simulink model "adrc_pid"  (R2025b)
settings: Solver=VariableStepAuto  StartTime=0.0  StopTime=50  RelTol=1e-3
values from neighbouring files (symbols this model uses):
  Alloc = [ kf,     kf,     kf,     kf ... (first row only)    [quad_params.m]
  Area = 2*L*Width    (= 0.072)    [quad_params.m]
  g = 9.81    [quad_params.m]
  h = [0 ... (first row only)    [Madgwick.m]    (also in quad_params.m = 0.2; umich_learning.m = x(:,1))
  h0 = Ts    (= 0.001)    [quad_params.m]
  inertia_mx = [Ixx; Iyy; Izz;]    [quad_params.m]
  init_h = 0.03    [quad_params.m]
  K_alloc = Alloc \ diag([W, 1, 1, 1])    [quad_params.m]
  max_rad_s_2 = max_rad_s ^ 2    (= 4279618.17072)    [quad_params.m]
  r0_position = 1    [quad_params.m]
  rho_air = 1.225    [quad_params.m]
  rho_water = 1000    [quad_params.m]
  Trot = 0.01    [quad_params.m]
  Ts = 0.001    [get_noise.m]    (also in quad_params.m; test.m = 0.002)
  W = 0.7 + 4*m_prop    (= 0.74)    [quad_params.m]
undefined symbols (not defined in the file or in its folder): adrcD
libraries: simulink x8
settings Model: Creator=David  LastModifiedBy=David

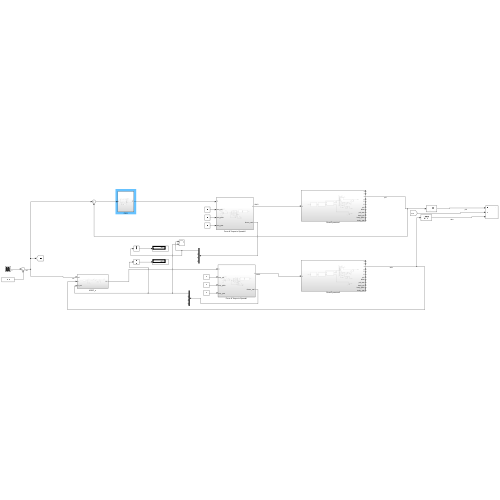
[thumbnail: Simulink's stored preview of the top-level diagram]
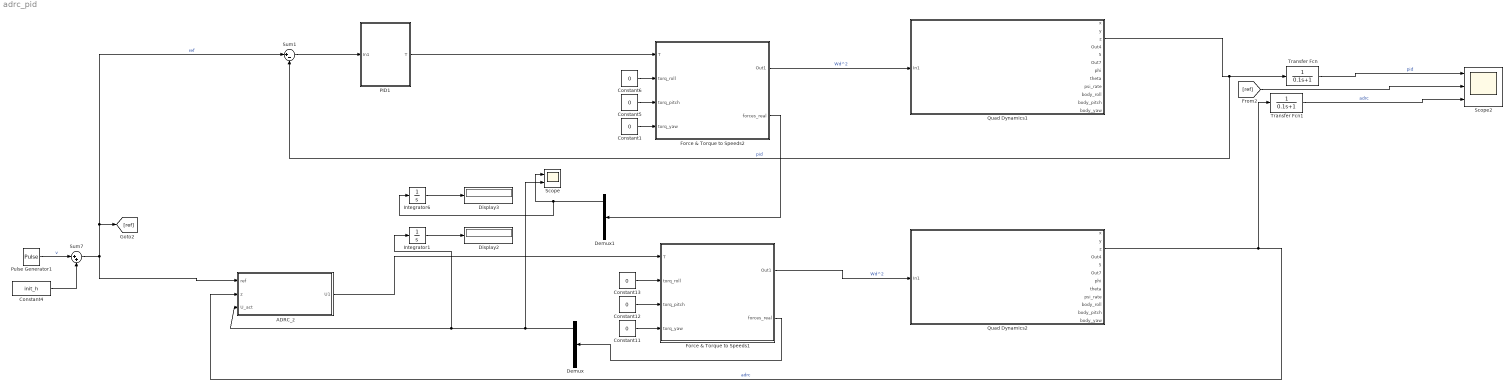
== system adrc_pid ==
  ADRC_z : Subsystem
  Constant{1,5..6,11..13} (6 alike) : Constant  Value=0
  Constant4 : Constant  Value=init_h
  Demux : Demux
  Demux1 : Demux
  Display2 : Display
  Display3 : Display
  Force & Torque to Speeds1 : Subsystem
  Force & Torque to Speeds2 : Subsystem
  Integrator1 : Integrator
  Integrator6 : Integrator
  PID1 : Subsystem
  Pulse Generator1 : DiscretePulseGenerator  PulseType=Time based  Period=30  PulseWidth=50  PhaseDelay=2
  Quad Dynamics1 : Subsystem
  Quad Dynamics2 : Subsystem
  Scope : Scope  NumInputPorts=2
      settings: ActiveDisplayYMinimum=-3.3627043852616136  ActiveDisplayYMaximum=30.264339467354532
  Scope2 : Scope  NumInputPorts=3
      settings: ActiveDisplayYMinimum=-0.12874999999999998  ActiveDisplayYMaximum=1.15875  DataLoggingVariableName=ScopeData2
  Sum1 : Sum  Inputs=|+-
  Sum7 : Sum  Inputs=|++
  Transfer Fcn : TransferFcn  Denominator=[0.1 1]
  Transfer Fcn1 : TransferFcn  Denominator=[0.1 1]
  wires:
  Integrator6/1 -> Display3/1
  Integrator1/1 -> Display2/1
  Pulse Generator1/1 -> Sum7/1  "v"
  ADRC_z/1(U1) -> Force & Torque to Speeds1/1(T)
  Constant4/1 -> Sum7/2
  Sum7/1 -> ADRC_z/1(ref), [ref], Sum1/1  "ref"
  Sum1/1 -> PID1/1(In1)
  PID1/1(T) -> Force & Torque to Speeds2/1(T)
  Constant11/1 -> Force & Torque to Speeds1/4(torq_yaw)
  Constant12/1 -> Force & Torque to Speeds1/3(torq_pitch)
  Constant13/1 -> Force & Torque to Speeds1/2(torq_roll)
  Quad Dynamics2/3(z) -> ADRC_z/2(z), Transfer Fcn1/1  "adrc"
  Constant1/1 -> Force & Torque to Speeds2/4(torq_yaw)
  Constant5/1 -> Force & Torque to Speeds2/3(torq_pitch)
  Constant6/1 -> Force & Torque to Speeds2/2(torq_roll)
  [ref] -> Scope2/2
  Force & Torque to Speeds2/1(Out1) -> Quad Dynamics1/1(In1)  "Wd^2"
  Force & Torque to Speeds1/1(Out1) -> Quad Dynamics2/1(In1)  "Wd^2"
  Force & Torque to Speeds1/2(forces_real) -> Demux/1
  Demux/1 -> Scope/2, Integrator1/1, ADRC_z/3(U_act)
  Quad Dynamics1/3(z) -> Sum1/2, Transfer Fcn/1  "pid"
  Transfer Fcn/1 -> Scope2/1  "pid"
  Transfer Fcn1/1 -> Scope2/3  "adrc"
  Force & Torque to Speeds2/2(forces_real) -> Demux1/1
  Demux1/1 -> Integrator6/1, Scope/1

== system adrc_pid/ADRC_z ==
  ref : Inport
  z : Inport  Port=2
  U_act : Inport  Port=3
  Constant : Constant  Value=adrcD.z.b0
  Constant1 : Constant  Commented=on  Value=g
  Divide : Product  Inputs=*/
  Gain : Gain  Gain=adrcD.z.k1
  Gain1 : Gain  Gain=1/W
  Gain2 : Gain  Gain=adrcD.z.k2
  Scope : Scope
      settings: ActiveDisplayYMinimum=-1  ActiveDisplayYMaximum=1  DataLoggingVariableName=ScopeData24
  Scope1 : Scope
      settings: ActiveDisplayYMinimum=-1  ActiveDisplayYMaximum=1  DataLoggingVariableName=ScopeData7
  Scope3 : Scope
      settings: ActiveDisplayYMinimum=-1  ActiveDisplayYMaximum=1  DataLoggingVariableName=ScopeData12
  Scope4 : Scope  NumInputPorts=2
      settings: ActiveDisplayYMinimum=-1  ActiveDisplayYMaximum=1  DataLoggingVariableName=ScopeData5
  Sum2 : Sum  Inputs=|+++
  Sum3 : Sum  Inputs=|++
  TD1 : Subsystem
  adrcD : Subsystem
  U1 : Outport
  wires:
  ref/1 -> TD1/1(v)
  TD1/1(ref) -> Gain/1, Scope/1
  Constant/1 -> Divide/2
  Gain/1 -> Sum2/1
  TD1/2(dref) -> Scope3/1, Gain2/1
  Gain2/1 -> Sum2/2
  Sum2/1 -> Scope1/1, Divide/1
  Constant1/1 -> Sum2/3
  Sum3/1 -> Gain1/1
  Gain1/1 -> Scope4/2, U1/1
  U_act/1 -> Scope4/1, adrcD/1(U_act)
  z/1 -> adrcD/2(y)
  adrcD/1(U) -> Sum3/2
  Divide/1 -> Sum3/1

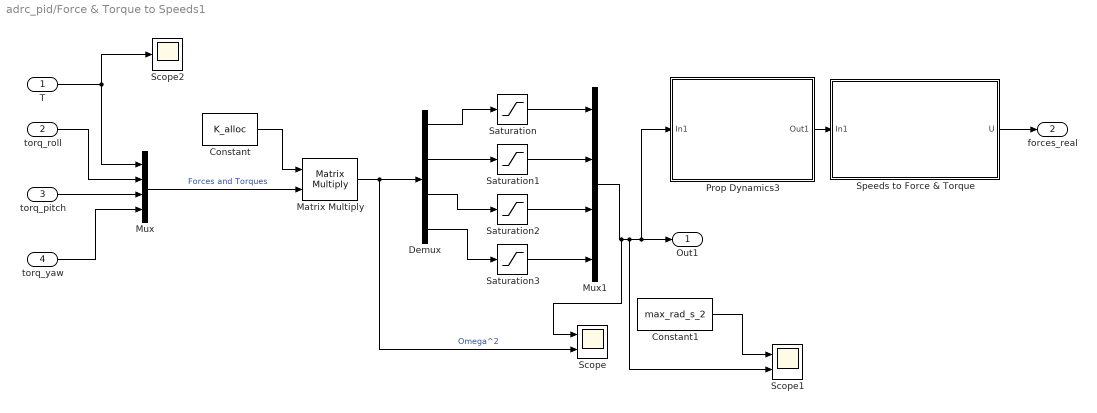
== system adrc_pid/Force & Torque to Speeds1 ==
  T : Inport
  torq_roll : Inport  Port=2
  torq_pitch : Inport  Port=3
  torq_yaw : Inport  Port=4
  Constant : Constant  Value=K_alloc
  Constant1 : Constant  Value=max_rad_s_2
  Demux : Demux
  Matrix Multiply : Product  Multiplication=Matrix(*)
  Mux : Mux
  Mux1 : Mux
  Prop Dynamics3 : Subsystem
  Saturation{,1..3} (4 alike) : Saturate  UpperLimit=max_rad_s_2  LowerLimit=0
  Scope : Scope  NumInputPorts=2
      settings: ActiveDisplayYMinimum=1.3835408867028086E+6  ActiveDisplayYMaximum=1.3836491858320688E+6  DataLoggingVariableName=ScopeData11
  Scope1 : Scope  NumInputPorts=2
      settings: ActiveDisplayYMinimum=-534952.27133938007  ActiveDisplayYMaximum=4.8145704420544216E+6  DataLoggingVariableName=ScopeData25
  Scope2 : Scope
      settings: ActiveDisplayYMinimum=-22.315254964417129  ActiveDisplayYMaximum=34.792796764645914  DataLoggingVariableName=ScopeData9
  Speeds to Force & Torque : Subsystem
  Out1 : Outport
  forces_real : Outport  Port=2
  wires:
  Matrix Multiply/1 -> Scope/2, Demux/1  "Omega^2"
  torq_yaw/1 -> Mux/4
  torq_pitch/1 -> Mux/3
  torq_roll/1 -> Mux/2
  T/1 -> Mux/1, Scope2/1
  Constant/1 -> Matrix Multiply/1
  Mux/1 -> Matrix Multiply/2  "Forces and Torques"
  Saturation3/1 -> Mux1/4
  Demux/4 -> Saturation3/1
  Demux/2 -> Saturation1/1
  Demux/1 -> Saturation/1
  Demux/3 -> Saturation2/1
  Saturation1/1 -> Mux1/2
  Saturation/1 -> Mux1/1
  Saturation2/1 -> Mux1/3
  Mux1/1 -> Scope/1, Scope1/2, Prop Dynamics3/1(In1), Out1/1
  Speeds to Force & Torque/1(U) -> forces_real/1
  Prop Dynamics3/1(Out1) -> Speeds to Force & Torque/1(In1)
  Constant1/1 -> Scope1/1

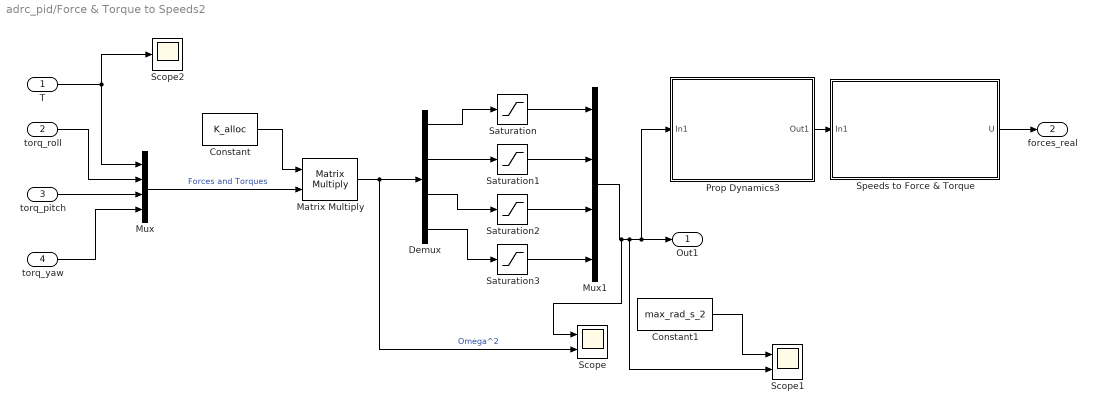
== system adrc_pid/Force & Torque to Speeds2 ==
  T : Inport
  torq_roll : Inport  Port=2
  torq_pitch : Inport  Port=3
  torq_yaw : Inport  Port=4
  Constant : Constant  Value=K_alloc
  Constant1 : Constant  Value=max_rad_s_2
  Demux : Demux
  Matrix Multiply : Product  Multiplication=Matrix(*)
  Mux : Mux
  Mux1 : Mux
  Prop Dynamics3 : Subsystem
  Saturation{,1..3} (4 alike) : Saturate  UpperLimit=max_rad_s_2  LowerLimit=0
  Scope : Scope  NumInputPorts=2
      settings: ActiveDisplayYMinimum=1.3835408867028086E+6  ActiveDisplayYMaximum=1.3836491858320688E+6  DataLoggingVariableName=ScopeData11
  Scope1 : Scope  NumInputPorts=2
      settings: ActiveDisplayYMinimum=-534952.27133938007  ActiveDisplayYMaximum=4.8145704420544216E+6  DataLoggingVariableName=ScopeData25
  Scope2 : Scope
      settings: ActiveDisplayYMinimum=-22.315254964417129  ActiveDisplayYMaximum=34.792796764645914  DataLoggingVariableName=ScopeData9
  Speeds to Force & Torque : Subsystem
  Out1 : Outport
  forces_real : Outport  Port=2
  wires:
  Constant1/1 -> Scope1/1
  Prop Dynamics3/1(Out1) -> Speeds to Force & Torque/1(In1)
  Speeds to Force & Torque/1(U) -> forces_real/1
  Mux1/1 -> Out1/1, Prop Dynamics3/1(In1), Scope1/2, Scope/1
  Saturation2/1 -> Mux1/3
  Saturation/1 -> Mux1/1
  Saturation1/1 -> Mux1/2
  Demux/3 -> Saturation2/1
  Demux/1 -> Saturation/1
  Demux/2 -> Saturation1/1
  Demux/4 -> Saturation3/1
  Saturation3/1 -> Mux1/4
  Mux/1 -> Matrix Multiply/2  "Forces and Torques"
  Constant/1 -> Matrix Multiply/1
  T/1 -> Scope2/1, Mux/1
  torq_roll/1 -> Mux/2
  torq_pitch/1 -> Mux/3
  torq_yaw/1 -> Mux/4
  Matrix Multiply/1 -> Demux/1, Scope/2  "Omega^2"

== system adrc_pid/PID1 ==
  In1 : Inport
  Gain : Gain  Gain=90
  Gain1 : Gain  Gain=20
  Gain2 : Gain  Gain=35
  Scope : Scope  NumInputPorts=3
      settings: ActiveDisplayYMinimum=-114.74585937242431  ActiveDisplayYMaximum=434.00912961546419  DataLoggingVariableName=ScopeData6
  Sum1 : Sum  Inputs=|+++
  Transfer Fcn : TransferFcn  Numerator=[1 0]  Denominator=[0.01 1]
  Transfer Fcn1 : TransferFcn  Denominator=[1 0]
  T : Outport
  wires:
  Sum1/1 -> T/1
  Transfer Fcn/1 -> Sum1/2, Scope/3  "D"
  Transfer Fcn1/1 -> Scope/1, Sum1/3  "I"
  Gain/1 -> Sum1/1, Scope/2  "P"
  Gain2/1 -> Transfer Fcn1/1
  Gain1/1 -> Transfer Fcn/1
  In1/1 -> Gain1/1, Gain/1, Gain2/1

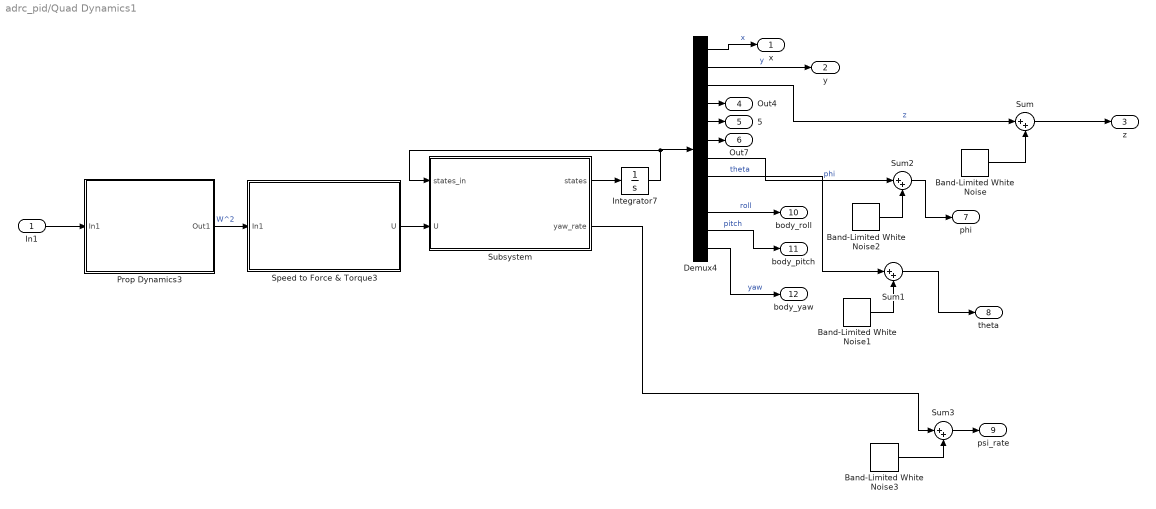
== system adrc_pid/Quad Dynamics1 ==
  In1 : Inport
  Band-Limited White Noise : simulink/Sources/Band-Limited White Noise  Cov=[2.6540e-06]  Ts=0.02  seed=[23341]
  Band-Limited White Noise1 : simulink/Sources/Band-Limited White Noise  Cov=[2e-6]  Ts=0.001  seed=[23342]
  Band-Limited White Noise2 : simulink/Sources/Band-Limited White Noise  Cov=[2e-6]  Ts=0.001  seed=[23341]
  Band-Limited White Noise3 : simulink/Sources/Band-Limited White Noise  Cov=[3.7430331138e-5]  Ts=0.001  seed=[23343]
  Demux4 : Demux  Outputs=12
  Integrator7 : Integrator  InitialCondition=zeros(12,1)
  Prop Dynamics3 : Subsystem
  Speed to Force & Torque3 : Subsystem
  Subsystem : Subsystem
  Sum{,1..3} (4 alike) : Sum  Inputs=|++
  x : Outport
  y : Outport  Port=2
  z : Outport  Port=3
  Out4 : Outport  Port=4
  5 : Outport  Port=5
  Out7 : Outport  Port=6
  phi : Outport  Port=7
  theta : Outport  Port=8
  psi_rate : Outport  Port=9
  body_roll : Outport  Port=10
  body_pitch : Outport  Port=11
  body_yaw : Outport  Port=12
  wires:
  Sum3/1 -> psi_rate/1
  Band-Limited White Noise3/1 -> Sum3/2
  Sum2/1 -> phi/1
  Band-Limited White Noise2/1 -> Sum2/2
  Sum1/1 -> theta/1
  Band-Limited White Noise1/1 -> Sum1/2
  Band-Limited White Noise/1 -> Sum/2
  Sum/1 -> z/1
  Subsystem/2(yaw_rate) -> Sum3/1
  In1/1 -> Prop Dynamics3/1(In1)
  Demux4/4 -> Out4/1
  Demux4/5 -> 5/1
  Demux4/6 -> Out7/1
  Demux4/12 -> body_yaw/1  "yaw"
  Demux4/11 -> body_pitch/1  "pitch"
  Demux4/8 -> Sum1/1  "theta"
  Demux4/3 -> Sum/1  "z"
  Demux4/7 -> Sum2/1  "phi"
  Demux4/10 -> body_roll/1  "roll"
  Integrator7/1 -> Subsystem/1(states_in), Demux4/1
  Speed to Force & Torque3/1(U) -> Subsystem/2(U)
  Subsystem/1(states) -> Integrator7/1
  Demux4/1 -> x/1  "x"
  Prop Dynamics3/1(Out1) -> Speed to Force & Torque3/1(In1)  "W^2"
  Demux4/2 -> y/1  "y"

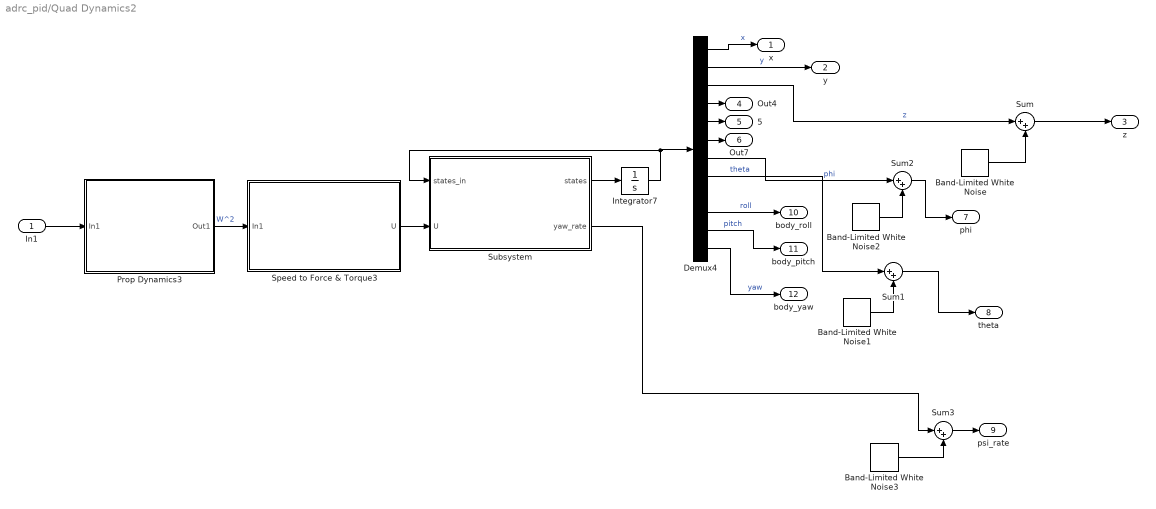
== system adrc_pid/Quad Dynamics2 ==
  In1 : Inport
  Band-Limited White Noise : simulink/Sources/Band-Limited White Noise  Cov=[2.6540e-06]  Ts=0.02  seed=[23341]
  Band-Limited White Noise1 : simulink/Sources/Band-Limited White Noise  Cov=[2e-6]  Ts=0.001  seed=[23342]
  Band-Limited White Noise2 : simulink/Sources/Band-Limited White Noise  Cov=[2e-6]  Ts=0.001  seed=[23341]
  Band-Limited White Noise3 : simulink/Sources/Band-Limited White Noise  Cov=[3.7430331138e-5]  Ts=0.001  seed=[23343]
  Demux4 : Demux  Outputs=12
  Integrator7 : Integrator  InitialCondition=zeros(12,1)
  Prop Dynamics3 : Subsystem
  Speed to Force & Torque3 : Subsystem
  Subsystem : Subsystem
  Sum{,1..3} (4 alike) : Sum  Inputs=|++
  x : Outport
  y : Outport  Port=2
  z : Outport  Port=3
  Out4 : Outport  Port=4
  5 : Outport  Port=5
  Out7 : Outport  Port=6
  phi : Outport  Port=7
  theta : Outport  Port=8
  psi_rate : Outport  Port=9
  body_roll : Outport  Port=10
  body_pitch : Outport  Port=11
  body_yaw : Outport  Port=12
  wires:
  Sum3/1 -> psi_rate/1
  Band-Limited White Noise3/1 -> Sum3/2
  Sum2/1 -> phi/1
  Band-Limited White Noise2/1 -> Sum2/2
  Sum1/1 -> theta/1
  Band-Limited White Noise1/1 -> Sum1/2
  Band-Limited White Noise/1 -> Sum/2
  Sum/1 -> z/1
  Subsystem/2(yaw_rate) -> Sum3/1
  In1/1 -> Prop Dynamics3/1(In1)
  Demux4/4 -> Out4/1
  Demux4/5 -> 5/1
  Demux4/6 -> Out7/1
  Demux4/12 -> body_yaw/1  "yaw"
  Demux4/11 -> body_pitch/1  "pitch"
  Demux4/8 -> Sum1/1  "theta"
  Demux4/3 -> Sum/1  "z"
  Demux4/7 -> Sum2/1  "phi"
  Demux4/10 -> body_roll/1  "roll"
  Integrator7/1 -> Subsystem/1(states_in), Demux4/1
  Speed to Force & Torque3/1(U) -> Subsystem/2(U)
  Subsystem/1(states) -> Integrator7/1
  Demux4/1 -> x/1  "x"
  Prop Dynamics3/1(Out1) -> Speed to Force & Torque3/1(In1)  "W^2"
  Demux4/2 -> y/1  "y"

== system adrc_pid/ADRC_z/TD1 ==
  v : Inport
  Constant11 : Constant  Value=r0_position
  Constant12 : Constant  Value=h0
  Delay One Step : Delay  DelayLength=1  SampleTime=Ts
  Delay One Step1 : Delay  DelayLength=1  SampleTime=Ts
  Gain3 : Gain  Gain=Ts
  Gain4 : Gain  Gain=Ts
  Sum1 : Sum  Inputs=|++
  Sum6 : Sum  Inputs=|++
  Sum7 : Sum  Inputs=|+-
  fhan : MATLAB Function  TreatAsAtomicUnit=on
  ref : Outport
  dref : Outport  Port=2
  wires:
  v/1 -> Sum7/2
  Constant12/1 -> fhan/4(h0)
  Sum7/1 -> fhan/1(e)
  Constant11/1 -> fhan/3(r0)
  Delay One Step1/1 -> fhan/2(v2), Sum6/2, Gain4/1  "v2(k)"
  Gain4/1 -> Sum1/2
  Sum1/1 -> ref/1, Delay One Step/1  "v1(k+1)"
  Sum6/1 -> dref/1, Delay One Step1/1  "v2(k+1)"
  Gain3/1 -> Sum6/1
  Delay One Step/1 -> Sum1/1, Sum7/1  "v1"
  fhan/1(u) -> Gain3/1

== system adrc_pid/ADRC_z/adrcD ==
  U_act : Inport
  y : Inport  Port=2
  Add : Sum  Inputs=-++-
  Add1 : Sum  Inputs=-++-
  Add2 : Sum  Inputs=+-
  Delay One Step : Delay  DelayLength=1  SampleTime=Ts
  Delay One Step1 : Delay  DelayLength=1  SampleTime=Ts
  Delay One Step2 : Delay  DelayLength=1  SampleTime=Ts
  Gain10 : Gain  Gain=adrcD.z.gamma1
  Gain11 : Gain  Gain=adrcD.z.gamma2
  Gain3 : Gain  Gain=adrcD.z.beta0
  Gain4 : Gain  Gain=adrcD.z.beta1
  Gain5 : Gain  Gain=adrcD.z.beta2
  Gain6 : Gain  Gain=adrcD.z.alpha3
  Gain7 : Gain  Gain=adrcD.z.alpha1
  Gain8 : Gain  Gain=adrcD.z.alpha2
  Gain9 : Gain  Gain=adrcD.z.gamma0
  Sum1 : Sum  Inputs=|+-
  U : Outport
  wires:
  Gain4/1 -> Add/1
  Gain8/1 -> Add1/4
  Add2/1 -> Delay One Step1/1
  y/1 -> Gain5/1, Gain4/1, Gain3/1
  U_act/1 -> Gain9/1, Gain11/1, Gain10/1
  Gain7/1 -> Add/4
  Gain11/1 -> Add2/1
  Gain3/1 -> Sum1/2
  Sum1/1 -> U/1, Gain6/1, Gain8/1, Gain7/1
  Add1/1 -> Delay One Step/1
  Gain5/1 -> Add1/1
  Gain10/1 -> Add1/2
  Add/1 -> Delay One Step2/1
  Gain9/1 -> Add/2
  Delay One Step1/1 -> Add1/3
  Delay One Step2/1 -> Sum1/1
  Gain6/1 -> Add2/2
  Delay One Step/1 -> Add/3

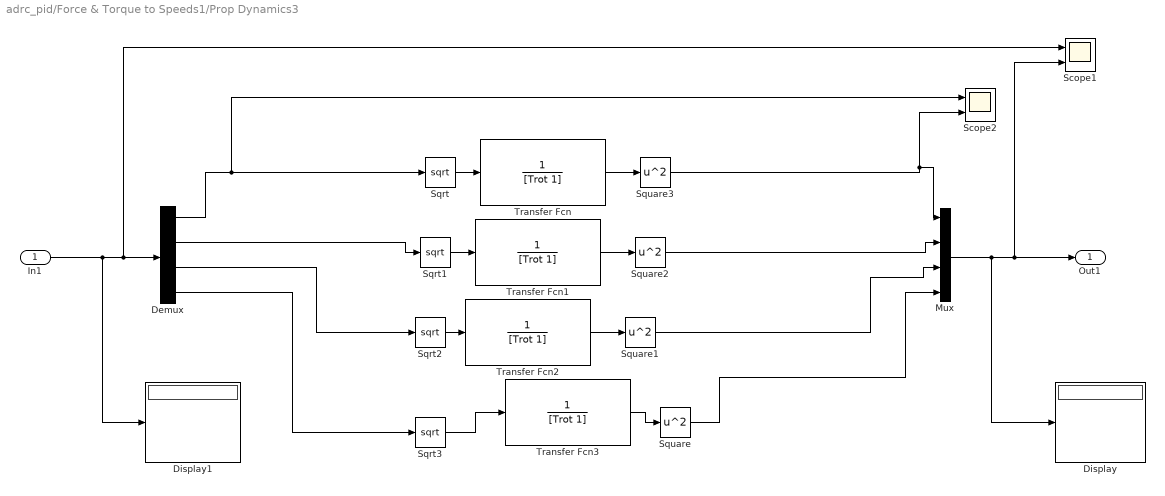
== system adrc_pid/Force & Torque to Speeds1/Prop Dynamics3 ==
  In1 : Inport
  Demux : Demux
  Display : Display
  Display1 : Display
  Mux : Mux
  Scope1 : Scope  NumInputPorts=2
      settings: ActiveDisplayYMinimum=112181.7837613984  ActiveDisplayYMaximum=826252.36344831332  DataLoggingVariableName=ScopeData22
  Scope2 : Scope  NumInputPorts=2
      settings: ActiveDisplayYMinimum=474145.79333634069  ActiveDisplayYMaximum=566090.11578068486  DataLoggingVariableName=ScopeData26
  Sqrt{,1..3} (4 alike) : Sqrt
  Square{,1..3} (4 alike) : Math  Operator=square
  Transfer Fcn{,1..3} (4 alike) : TransferFcn  Denominator=[Trot 1]
  Out1 : Outport
  wires:
  Square/1 -> Mux/4
  Demux/4 -> Sqrt3/1
  Demux/3 -> Sqrt2/1
  Demux/2 -> Sqrt1/1
  Demux/1 -> Sqrt/1, Scope2/1
  Sqrt3/1 -> Transfer Fcn3/1
  Sqrt2/1 -> Transfer Fcn2/1
  Sqrt1/1 -> Transfer Fcn1/1
  Sqrt/1 -> Transfer Fcn/1
  Transfer Fcn3/1 -> Square/1
  Transfer Fcn2/1 -> Square1/1
  Transfer Fcn/1 -> Square3/1
  Transfer Fcn1/1 -> Square2/1
  Mux/1 -> Scope1/2, Out1/1, Display/1
  In1/1 -> Scope1/1, Demux/1, Display1/1
  Square3/1 -> Scope2/2, Mux/1
  Square2/1 -> Mux/2
  Square1/1 -> Mux/3

== system adrc_pid/Force & Torque to Speeds1/Speeds to Force & Torque ==
  In1 : Inport
  Constant1 : Constant  Value=Alloc
  Matrix Multiply1 : Product  Multiplication=Matrix(*)
  U : Outport
  wires:
  Constant1/1 -> Matrix Multiply1/1
  Matrix Multiply1/1 -> U/1
  In1/1 -> Matrix Multiply1/2  "Omega^2"

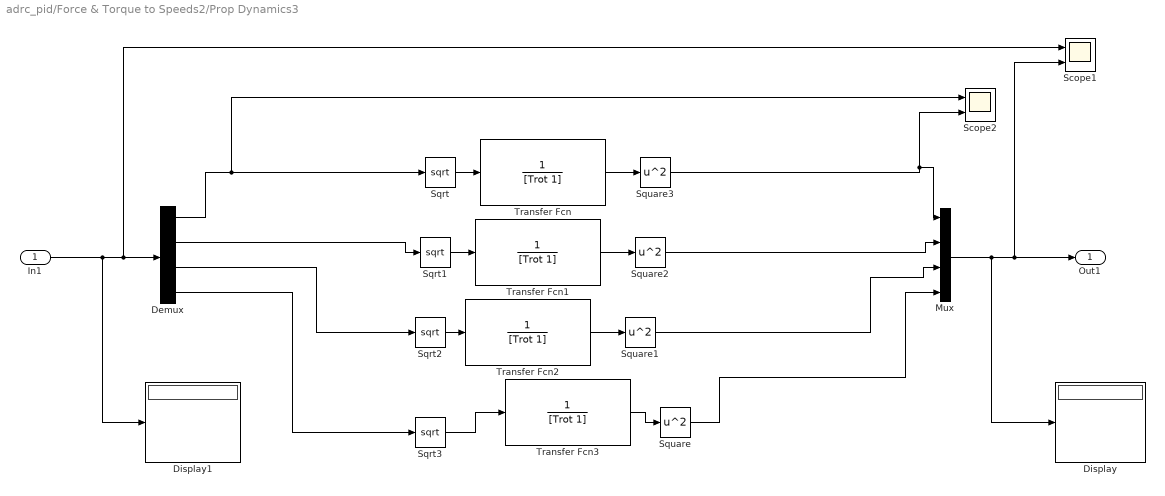
== system adrc_pid/Force & Torque to Speeds2/Prop Dynamics3 ==
  In1 : Inport
  Demux : Demux
  Display : Display
  Display1 : Display
  Mux : Mux
  Scope1 : Scope  NumInputPorts=2
      settings: ActiveDisplayYMinimum=112181.7837613984  ActiveDisplayYMaximum=826252.36344831332  DataLoggingVariableName=ScopeData22
  Scope2 : Scope  NumInputPorts=2
      settings: ActiveDisplayYMinimum=474145.79333634069  ActiveDisplayYMaximum=566090.11578068486  DataLoggingVariableName=ScopeData26
  Sqrt{,1..3} (4 alike) : Sqrt
  Square{,1..3} (4 alike) : Math  Operator=square
  Transfer Fcn{,1..3} (4 alike) : TransferFcn  Denominator=[Trot 1]
  Out1 : Outport
  wires:
  Square1/1 -> Mux/3
  Square2/1 -> Mux/2
  Square3/1 -> Mux/1, Scope2/2
  In1/1 -> Display1/1, Demux/1, Scope1/1
  Mux/1 -> Display/1, Out1/1, Scope1/2
  Transfer Fcn1/1 -> Square2/1
  Transfer Fcn/1 -> Square3/1
  Transfer Fcn2/1 -> Square1/1
  Transfer Fcn3/1 -> Square/1
  Sqrt/1 -> Transfer Fcn/1
  Sqrt1/1 -> Transfer Fcn1/1
  Sqrt2/1 -> Transfer Fcn2/1
  Sqrt3/1 -> Transfer Fcn3/1
  Demux/1 -> Scope2/1, Sqrt/1
  Demux/2 -> Sqrt1/1
  Demux/3 -> Sqrt2/1
  Demux/4 -> Sqrt3/1
  Square/1 -> Mux/4

== system adrc_pid/Force & Torque to Speeds2/Speeds to Force & Torque ==
  In1 : Inport
  Constant1 : Constant  Value=Alloc
  Matrix Multiply1 : Product  Multiplication=Matrix(*)
  U : Outport
  wires:
  In1/1 -> Matrix Multiply1/2  "Omega^2"
  Matrix Multiply1/1 -> U/1
  Constant1/1 -> Matrix Multiply1/1

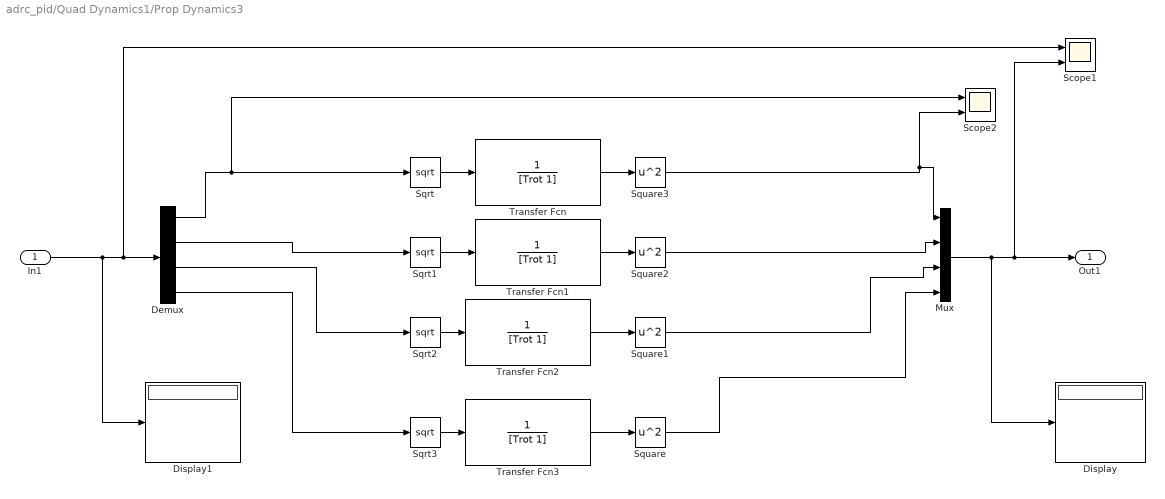
== system adrc_pid/Quad Dynamics1/Prop Dynamics3 ==
  In1 : Inport
  Demux : Demux
  Display : Display
  Display1 : Display
  Mux : Mux
  Scope1 : Scope  NumInputPorts=2
      settings: ActiveDisplayYMinimum=-75977.2512965213  ActiveDisplayYMaximum=683795.26166869176  DataLoggingVariableName=ScopeData22
  Scope2 : Scope  NumInputPorts=2
      settings: ActiveDisplayYMinimum=-75859.286983978411  ActiveDisplayYMaximum=682733.58285580587  DataLoggingVariableName=ScopeData26
  Sqrt{,1..3} (4 alike) : Sqrt
  Square{,1..3} (4 alike) : Math  Operator=square
  Transfer Fcn{,1..3} (4 alike) : TransferFcn  Denominator=[Trot 1]
  Out1 : Outport
  wires:
  Square1/1 -> Mux/3
  Square2/1 -> Mux/2
  Square3/1 -> Mux/1, Scope2/2
  In1/1 -> Display1/1, Demux/1, Scope1/1
  Mux/1 -> Display/1, Out1/1, Scope1/2
  Transfer Fcn1/1 -> Square2/1
  Transfer Fcn/1 -> Square3/1
  Transfer Fcn2/1 -> Square1/1
  Transfer Fcn3/1 -> Square/1
  Sqrt/1 -> Transfer Fcn/1
  Sqrt1/1 -> Transfer Fcn1/1
  Sqrt2/1 -> Transfer Fcn2/1
  Sqrt3/1 -> Transfer Fcn3/1
  Demux/1 -> Scope2/1, Sqrt/1
  Demux/2 -> Sqrt1/1
  Demux/3 -> Sqrt2/1
  Demux/4 -> Sqrt3/1
  Square/1 -> Mux/4

== system adrc_pid/Quad Dynamics1/Speed to Force & Torque3 ==
  In1 : Inport
  Constant1 : Constant  Value=Alloc
  Matrix Multiply1 : Product  Multiplication=Matrix(*)
  U : Outport
  wires:
  In1/1 -> Matrix Multiply1/2  "Omega^2"
  Matrix Multiply1/1 -> U/1
  Constant1/1 -> Matrix Multiply1/1

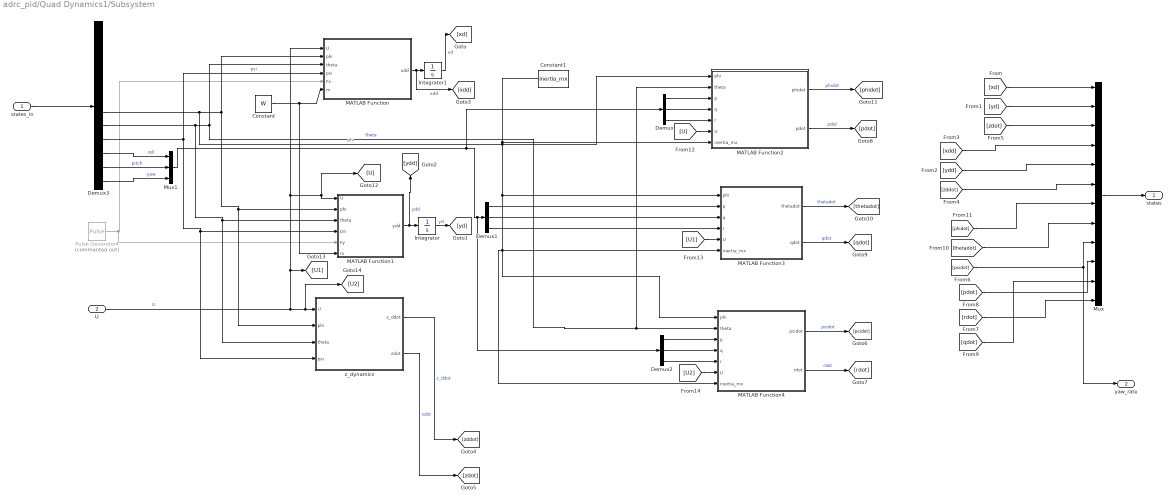
== system adrc_pid/Quad Dynamics1/Subsystem ==
  states_in : Inport
  U : Inport  Port=2
  Constant : Constant  Value=W
  Constant1 : Constant  Value=inertia_mx
  Demux : Demux  Outputs=3
  Demux1 : Demux  Outputs=3
  Demux2 : Demux  Outputs=3
  Demux3 : Demux  Outputs=12
  Integrator : Integrator
  Integrator1 : Integrator
  MATLAB Function : MATLAB Function  TreatAsAtomicUnit=on
  MATLAB Function1 : MATLAB Function  TreatAsAtomicUnit=on
  MATLAB Function2 : MATLAB Function  TreatAsAtomicUnit=on
  MATLAB Function3 : MATLAB Function  TreatAsAtomicUnit=on
  MATLAB Function4 : MATLAB Function  TreatAsAtomicUnit=on
  Mux : Mux  Inputs=12
  Mux1 : Mux  Inputs=3
  Pulse Generator4 : DiscretePulseGenerator  Commented=on  PulseType=Time based  Amplitude=0.1  Period=5  PulseWidth=30  PhaseDelay=6
  z_dynamics : Subsystem
  states : Outport
  yaw_rate : Outport  Port=2
  wires:
  Pulse Generator4/1 -> MATLAB Function/5(Fx), MATLAB Function1/5(Fy)
  [U2] -> MATLAB Function4/6(U)
  [U1] -> MATLAB Function3/5(U)
  [U] -> MATLAB Function2/6(U)
  [phidot] -> Mux/7
  MATLAB Function2/1(phidot) -> [phidot]  "phidot"
  [thetadot] -> Mux/8
  MATLAB Function3/1(thetadot) -> [thetadot]  "thetadot"
  [qdot] -> Mux/11
  MATLAB Function3/2(qdot) -> [qdot]  "qdot"
  [pdot] -> Mux/10
  MATLAB Function2/2(pdot) -> [pdot]  "pdot"
  [rdot] -> Mux/12
  MATLAB Function4/2(rdot) -> [rdot]  "rdot"
  [psidot] -> yaw_rate/1, Mux/9
  MATLAB Function4/1(psidot) -> [psidot]  "psidot"
  [zdot] -> Mux/3
  z_dynamics/2(zdot) -> [zdot]  "zdot"
  [zddot] -> Mux/6
  z_dynamics/1(z_ddot) -> [zddot]  "z_ddot"
  [xdd] -> Mux/4
  [ydd] -> Mux/5
  [yd] -> Mux/2
  Integrator/1 -> [yd]  "yd"
  [xd] -> Mux/1
  Integrator1/1 -> [xd]  "xd"
  Demux/3 -> MATLAB Function2/5(r)
  Demux/2 -> MATLAB Function2/4(q)
  Demux/1 -> MATLAB Function2/3(p)
  Demux2/3 -> MATLAB Function4/5(r)
  Demux2/2 -> MATLAB Function4/4(q)
  Demux2/1 -> MATLAB Function4/3(p)
  Demux1/3 -> MATLAB Function3/4(r)
  Demux1/2 -> MATLAB Function3/3(q)
  Demux1/1 -> MATLAB Function3/2(p)
  Mux1/1 -> Demux1/1, Demux2/1, Demux/1
  Demux3/10 -> Mux1/1  "roll"
  Demux3/12 -> Mux1/3  "yaw"
  Demux3/11 -> Mux1/2  "pitch"
  Constant1/1 -> MATLAB Function2/7(inertia_mx), MATLAB Function3/6(inertia_mx), MATLAB Function4/7(inertia_mx)
  Constant/1 -> MATLAB Function1/6(m), MATLAB Function/6(m)
  Demux3/9 -> MATLAB Function/4(psi), MATLAB Function1/4(psi), z_dynamics/4(psi)  "psi"
  Demux3/8 -> MATLAB Function/3(theta), MATLAB Function4/2(theta), MATLAB Function2/2(theta), MATLAB Function1/3(theta), z_dynamics/3(theta)  "theta"
  Demux3/7 -> MATLAB Function1/2(phi), z_dynamics/2(phi), MATLAB Function/2(phi), MATLAB Function2/1(phi), MATLAB Function4/1(phi), MATLAB Function3/1(phi)  "phi"
  U/1 -> [U1], MATLAB Function1/1(U), [U], MATLAB Function/1(U), z_dynamics/1(U), [U2]  "U"
  states_in/1 -> Demux3/1
  Mux/1 -> states/1
  MATLAB Function1/1(ydd) -> Integrator/1, [ydd]  "ydd"
  MATLAB Function/1(xdd) -> Integrator1/1, [xdd]  "xdd"

== system adrc_pid/Quad Dynamics2/Prop Dynamics3 ==
  In1 : Inport
  Demux : Demux
  Display : Display
  Display1 : Display
  Mux : Mux
  Scope1 : Scope  NumInputPorts=2
      settings: ActiveDisplayYMinimum=-75977.2512965213  ActiveDisplayYMaximum=683795.26166869176  DataLoggingVariableName=ScopeData22
  Scope2 : Scope  NumInputPorts=2
      settings: ActiveDisplayYMinimum=-75859.286983978411  ActiveDisplayYMaximum=682733.58285580587  DataLoggingVariableName=ScopeData26
  Sqrt{,1..3} (4 alike) : Sqrt
  Square{,1..3} (4 alike) : Math  Operator=square
  Transfer Fcn{,1..3} (4 alike) : TransferFcn  Denominator=[Trot 1]
  Out1 : Outport
  wires:
  Square1/1 -> Mux/3
  Square2/1 -> Mux/2
  Square3/1 -> Mux/1, Scope2/2
  In1/1 -> Display1/1, Demux/1, Scope1/1
  Mux/1 -> Display/1, Out1/1, Scope1/2
  Transfer Fcn1/1 -> Square2/1
  Transfer Fcn/1 -> Square3/1
  Transfer Fcn2/1 -> Square1/1
  Transfer Fcn3/1 -> Square/1
  Sqrt/1 -> Transfer Fcn/1
  Sqrt1/1 -> Transfer Fcn1/1
  Sqrt2/1 -> Transfer Fcn2/1
  Sqrt3/1 -> Transfer Fcn3/1
  Demux/1 -> Scope2/1, Sqrt/1
  Demux/2 -> Sqrt1/1
  Demux/3 -> Sqrt2/1
  Demux/4 -> Sqrt3/1
  Square/1 -> Mux/4

== system adrc_pid/Quad Dynamics2/Speed to Force & Torque3 ==
  In1 : Inport
  Constant1 : Constant  Value=Alloc
  Matrix Multiply1 : Product  Multiplication=Matrix(*)
  U : Outport
  wires:
  In1/1 -> Matrix Multiply1/2  "Omega^2"
  Matrix Multiply1/1 -> U/1
  Constant1/1 -> Matrix Multiply1/1

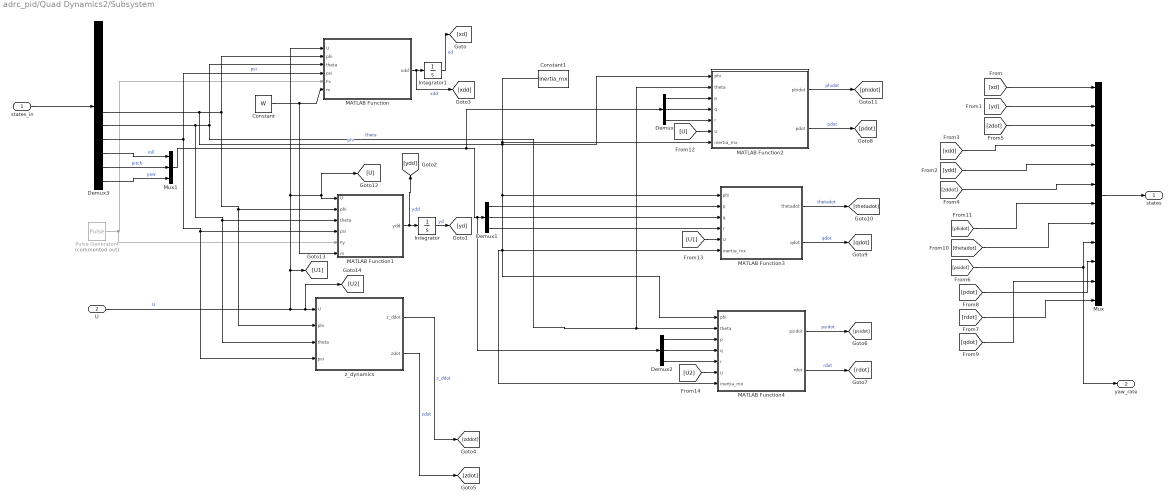
== system adrc_pid/Quad Dynamics2/Subsystem ==
  states_in : Inport
  U : Inport  Port=2
  Constant : Constant  Value=W
  Constant1 : Constant  Value=inertia_mx
  Demux : Demux  Outputs=3
  Demux1 : Demux  Outputs=3
  Demux2 : Demux  Outputs=3
  Demux3 : Demux  Outputs=12
  Integrator : Integrator
  Integrator1 : Integrator
  MATLAB Function : MATLAB Function  TreatAsAtomicUnit=on
  MATLAB Function1 : MATLAB Function  TreatAsAtomicUnit=on
  MATLAB Function2 : MATLAB Function  TreatAsAtomicUnit=on
  MATLAB Function3 : MATLAB Function  TreatAsAtomicUnit=on
  MATLAB Function4 : MATLAB Function  TreatAsAtomicUnit=on
  Mux : Mux  Inputs=12
  Mux1 : Mux  Inputs=3
  Pulse Generator4 : DiscretePulseGenerator  Commented=on  PulseType=Time based  Amplitude=0.1  Period=5  PulseWidth=30  PhaseDelay=6
  z_dynamics : Subsystem
  states : Outport
  yaw_rate : Outport  Port=2
  wires:
  Pulse Generator4/1 -> MATLAB Function/5(Fx), MATLAB Function1/5(Fy)
  [U2] -> MATLAB Function4/6(U)
  [U1] -> MATLAB Function3/5(U)
  [U] -> MATLAB Function2/6(U)
  [phidot] -> Mux/7
  MATLAB Function2/1(phidot) -> [phidot]  "phidot"
  [thetadot] -> Mux/8
  MATLAB Function3/1(thetadot) -> [thetadot]  "thetadot"
  [qdot] -> Mux/11
  MATLAB Function3/2(qdot) -> [qdot]  "qdot"
  [pdot] -> Mux/10
  MATLAB Function2/2(pdot) -> [pdot]  "pdot"
  [rdot] -> Mux/12
  MATLAB Function4/2(rdot) -> [rdot]  "rdot"
  [psidot] -> yaw_rate/1, Mux/9
  MATLAB Function4/1(psidot) -> [psidot]  "psidot"
  [zdot] -> Mux/3
  z_dynamics/2(zdot) -> [zdot]  "zdot"
  [zddot] -> Mux/6
  z_dynamics/1(z_ddot) -> [zddot]  "z_ddot"
  [xdd] -> Mux/4
  [ydd] -> Mux/5
  [yd] -> Mux/2
  Integrator/1 -> [yd]  "yd"
  [xd] -> Mux/1
  Integrator1/1 -> [xd]  "xd"
  Demux/3 -> MATLAB Function2/5(r)
  Demux/2 -> MATLAB Function2/4(q)
  Demux/1 -> MATLAB Function2/3(p)
  Demux2/3 -> MATLAB Function4/5(r)
  Demux2/2 -> MATLAB Function4/4(q)
  Demux2/1 -> MATLAB Function4/3(p)
  Demux1/3 -> MATLAB Function3/4(r)
  Demux1/2 -> MATLAB Function3/3(q)
  Demux1/1 -> MATLAB Function3/2(p)
  Mux1/1 -> Demux1/1, Demux2/1, Demux/1
  Demux3/10 -> Mux1/1  "roll"
  Demux3/12 -> Mux1/3  "yaw"
  Demux3/11 -> Mux1/2  "pitch"
  Constant1/1 -> MATLAB Function2/7(inertia_mx), MATLAB Function3/6(inertia_mx), MATLAB Function4/7(inertia_mx)
  Constant/1 -> MATLAB Function1/6(m), MATLAB Function/6(m)
  Demux3/9 -> MATLAB Function/4(psi), MATLAB Function1/4(psi), z_dynamics/4(psi)  "psi"
  Demux3/8 -> MATLAB Function/3(theta), MATLAB Function4/2(theta), MATLAB Function2/2(theta), MATLAB Function1/3(theta), z_dynamics/3(theta)  "theta"
  Demux3/7 -> MATLAB Function1/2(phi), z_dynamics/2(phi), MATLAB Function/2(phi), MATLAB Function2/1(phi), MATLAB Function4/1(phi), MATLAB Function3/1(phi)  "phi"
  U/1 -> [U1], MATLAB Function1/1(U), [U], MATLAB Function/1(U), z_dynamics/1(U), [U2]  "U"
  states_in/1 -> Demux3/1
  Mux/1 -> states/1
  MATLAB Function1/1(ydd) -> Integrator/1, [ydd]  "ydd"
  MATLAB Function/1(xdd) -> Integrator1/1, [xdd]  "xdd"

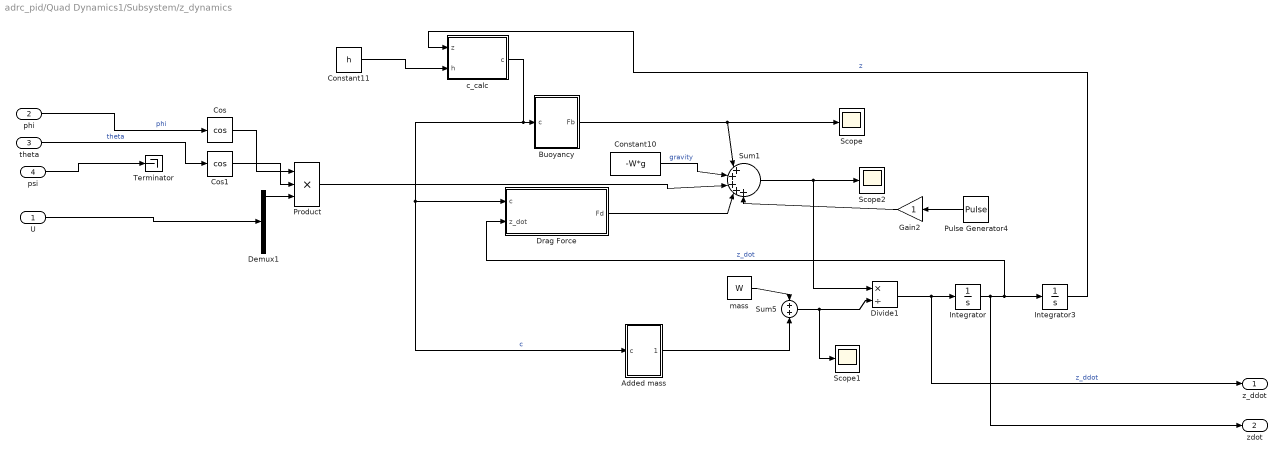
== system adrc_pid/Quad Dynamics1/Subsystem/z_dynamics ==
  U : Inport
  phi : Inport  Port=2
  theta : Inport  Port=3
  psi : Inport  Port=4
  Added mass : Subsystem
  Buoyancy : Subsystem
  Constant10 : Constant  Value=-W*g
  Constant11 : Constant  Value=h
  Cos : Trigonometry  Operator=cos
  Cos1 : Trigonometry  Operator=cos
  Demux1 : Demux
  Divide1 : Product  Inputs=*/
  Drag Force : Subsystem
  Gain2 : Gain
  Integrator : Integrator
  Integrator3 : Integrator
  Product : Product  Inputs=3
  Pulse Generator4 : DiscretePulseGenerator  PulseType=Time based  Amplitude=5  Period=5  PulseWidth=30  PhaseDelay=5
  Scope : Scope
      settings: ActiveDisplayYMinimum=3.324205069659222  ActiveDisplayYMaximum=24.046643881148977  DataLoggingVariableName=ScopeData4
  Scope1 : Scope
      settings: ActiveDisplayYMinimum=1.2962500000000001  ActiveDisplayYMaximum=1.7337500000000001  DataLoggingVariableName=ScopeData8
  Scope2 : Scope
      settings: ActiveDisplayYMinimum=-2.7468  ActiveDisplayYMaximum=24.721200000000003  DataLoggingVariableName=ScopeData10
  Sum1 : Sum  Inputs=|+++++
  Sum5 : Sum
  Terminator : Terminator
  c_calc : MATLAB Function  TreatAsAtomicUnit=on
  mass : Constant  Value=W
  z_ddot : Outport
  zdot : Outport  Port=2
  wires:
  Gain2/1 -> Sum1/5
  Pulse Generator4/1 -> Gain2/1
  U/1 -> Demux1/1
  Constant11/1 -> c_calc/2(h)
  Constant10/1 -> Sum1/2  "gravity"
  Buoyancy/1(Fb) -> Scope/1, Sum1/1
  Divide1/1 -> Integrator/1, z_ddot/1  "z_ddot"
  Drag Force/1(Fd) -> Sum1/4
  Integrator/1 -> zdot/1, Integrator3/1, Drag Force/2(z_dot)  "z_dot"
  Integrator3/1 -> c_calc/1(z)  "z"
  Sum5/1 -> Divide1/2, Scope1/1
  mass/1 -> Sum5/1
  Added mass/1(m_a) -> Sum5/2
  Product/1 -> Sum1/3
  c_calc/1(c) -> Buoyancy/1(c), Drag Force/1(c), Added mass/1(c)  "c"
  Sum1/1 -> Divide1/1, Scope2/1
  psi/1 -> Terminator/1
  Demux1/1 -> Product/3
  Cos1/1 -> Product/2
  Cos/1 -> Product/1
  theta/1 -> Cos1/1  "theta"
  phi/1 -> Cos/1  "phi"

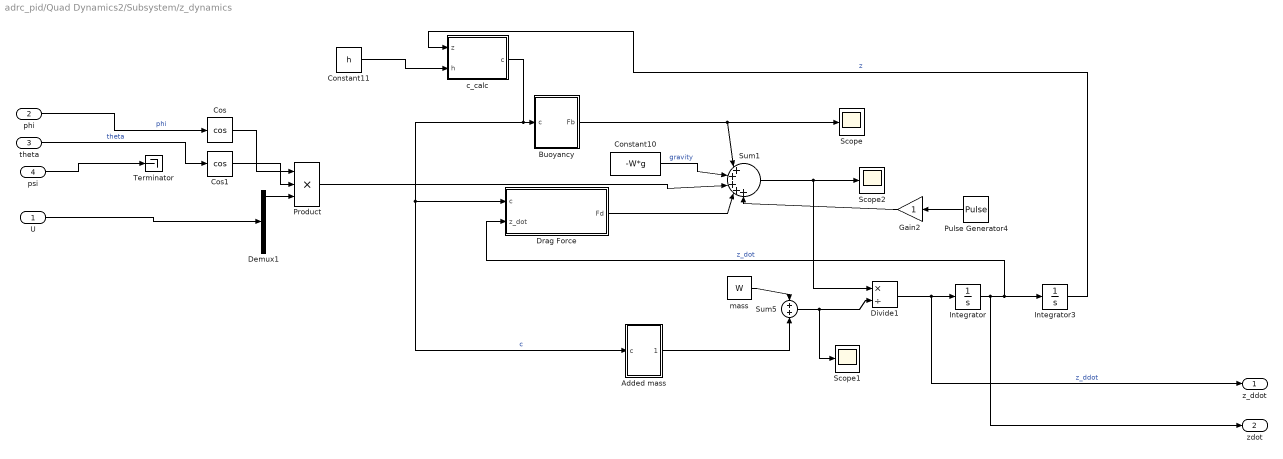
== system adrc_pid/Quad Dynamics2/Subsystem/z_dynamics ==
  U : Inport
  phi : Inport  Port=2
  theta : Inport  Port=3
  psi : Inport  Port=4
  Added mass : Subsystem
  Buoyancy : Subsystem
  Constant10 : Constant  Value=-W*g
  Constant11 : Constant  Value=h
  Cos : Trigonometry  Operator=cos
  Cos1 : Trigonometry  Operator=cos
  Demux1 : Demux
  Divide1 : Product  Inputs=*/
  Drag Force : Subsystem
  Gain2 : Gain
  Integrator : Integrator
  Integrator3 : Integrator
  Product : Product  Inputs=3
  Pulse Generator4 : DiscretePulseGenerator  PulseType=Time based  Amplitude=5  Period=5  PulseWidth=30  PhaseDelay=5
  Scope : Scope
      settings: ActiveDisplayYMinimum=3.324205069659222  ActiveDisplayYMaximum=24.046643881148977  DataLoggingVariableName=ScopeData4
  Scope1 : Scope
      settings: ActiveDisplayYMinimum=1.2962500000000001  ActiveDisplayYMaximum=1.7337500000000001  DataLoggingVariableName=ScopeData8
  Scope2 : Scope
      settings: ActiveDisplayYMinimum=-2.7468  ActiveDisplayYMaximum=24.721200000000003  DataLoggingVariableName=ScopeData10
  Sum1 : Sum  Inputs=|+++++
  Sum5 : Sum
  Terminator : Terminator
  c_calc : MATLAB Function  TreatAsAtomicUnit=on
  mass : Constant  Value=W
  z_ddot : Outport
  zdot : Outport  Port=2
  wires:
  Gain2/1 -> Sum1/5
  Pulse Generator4/1 -> Gain2/1
  U/1 -> Demux1/1
  Constant11/1 -> c_calc/2(h)
  Constant10/1 -> Sum1/2  "gravity"
  Buoyancy/1(Fb) -> Scope/1, Sum1/1
  Divide1/1 -> Integrator/1, z_ddot/1  "z_ddot"
  Drag Force/1(Fd) -> Sum1/4
  Integrator/1 -> zdot/1, Integrator3/1, Drag Force/2(z_dot)  "z_dot"
  Integrator3/1 -> c_calc/1(z)  "z"
  Sum5/1 -> Divide1/2, Scope1/1
  mass/1 -> Sum5/1
  Added mass/1(m_a) -> Sum5/2
  Product/1 -> Sum1/3
  c_calc/1(c) -> Buoyancy/1(c), Drag Force/1(c), Added mass/1(c)  "c"
  Sum1/1 -> Divide1/1, Scope2/1
  psi/1 -> Terminator/1
  Demux1/1 -> Product/3
  Cos1/1 -> Product/2
  Cos/1 -> Product/1
  theta/1 -> Cos1/1  "theta"
  phi/1 -> Cos/1  "phi"

== system adrc_pid/Quad Dynamics1/Subsystem/z_dynamics/Added mass ==
  c : Inport
  Product1 : Product
  added_mass : Constant  Value=0.05*rho_water
  m_a : Outport
  wires:
  c/1 -> Product1/2
  Product1/1 -> m_a/1
  added_mass/1 -> Product1/1

== system adrc_pid/Quad Dynamics1/Subsystem/z_dynamics/Buoyancy ==
  c : Inport
  Constant1 : Constant  Value=rho_water*Area*g
  Product : Product
  Fb : Outport
  wires:
  Product/1 -> Fb/1  "buoyancy"
  c/1 -> Product/1
  Constant1/1 -> Product/2

== system adrc_pid/Quad Dynamics1/Subsystem/z_dynamics/Drag Force ==
  c : Inport
  z_dot : Inport  Port=2
  Abs : Abs  SaturateOnIntegerOverflow=off
  Constant : Constant  Value=h
  Constant10 : Constant
  Constant11 : Constant  Value=Area
  Constant7 : Constant  Value=rho_air
  Constant8 : Constant  Value=rho_water
  Constant9 : Constant  Value=-0.5
  Divide : Product  Inputs=*/
  Product3 : Product
  Product4 : Product
  Product5 : Product  Inputs=5
  Sum2 : Sum
  Sum3 : Sum  Inputs=+-
  Fd : Outport
  wires:
  Constant/1 -> Divide/2
  c/1 -> Divide/1
  Constant7/1 -> Product3/1  "air"
  Product3/1 -> Sum2/1  "air drag"
  Abs/1 -> Product5/4
  z_dot/1 -> Product5/3, Abs/1
  Constant9/1 -> Product5/2
  Sum2/1 -> Product5/1
  Constant10/1 -> Sum3/1
  Constant8/1 -> Product4/1  "water"
  Sum3/1 -> Product3/2
  Constant11/1 -> Product5/5
  Product4/1 -> Sum2/2  "water drag"
  Product5/1 -> Fd/1  "drag force"
  Divide/1 -> Product4/2, Sum3/2

== system adrc_pid/Quad Dynamics2/Subsystem/z_dynamics/Added mass ==
  c : Inport
  Product1 : Product
  added_mass : Constant  Value=0.05*rho_water
  m_a : Outport
  wires:
  c/1 -> Product1/2
  Product1/1 -> m_a/1
  added_mass/1 -> Product1/1

== system adrc_pid/Quad Dynamics2/Subsystem/z_dynamics/Buoyancy ==
  c : Inport
  Constant1 : Constant  Value=rho_water*Area*g
  Product : Product
  Fb : Outport
  wires:
  Product/1 -> Fb/1  "buoyancy"
  c/1 -> Product/1
  Constant1/1 -> Product/2

== system adrc_pid/Quad Dynamics2/Subsystem/z_dynamics/Drag Force ==
  c : Inport
  z_dot : Inport  Port=2
  Abs : Abs  SaturateOnIntegerOverflow=off
  Constant : Constant  Value=h
  Constant10 : Constant
  Constant11 : Constant  Value=Area
  Constant7 : Constant  Value=rho_air
  Constant8 : Constant  Value=rho_water
  Constant9 : Constant  Value=-0.5
  Divide : Product  Inputs=*/
  Product3 : Product
  Product4 : Product
  Product5 : Product  Inputs=5
  Sum2 : Sum
  Sum3 : Sum  Inputs=+-
  Fd : Outport
  wires:
  Constant/1 -> Divide/2
  c/1 -> Divide/1
  Constant7/1 -> Product3/1  "air"
  Product3/1 -> Sum2/1  "air drag"
  Abs/1 -> Product5/4
  z_dot/1 -> Product5/3, Abs/1
  Constant9/1 -> Product5/2
  Sum2/1 -> Product5/1
  Constant10/1 -> Sum3/1
  Constant8/1 -> Product4/1  "water"
  Sum3/1 -> Product3/2
  Constant11/1 -> Product5/5
  Product4/1 -> Sum2/2  "water drag"
  Product5/1 -> Fd/1  "drag force"
  Divide/1 -> Product4/2, Sum3/2

== matlab function adrc_pid/Quad Dynamics2/Subsystem/MATLAB Function1 ==
  data: U input; ydd output; phi input; theta input; psi input; Fy input; m input
function ydd = y_dynamics(U, phi, theta, psi, Fy, m)

T = U(1);

ydd = (T/m)*(sin(psi)*sin(theta)*cos(phi) ...
               - cos(psi)*sin(phi)) + Fy/m;

end

== matlab function adrc_pid/ADRC_z/TD1/fhan ==
  data: e input; u output; v2 input; r0 input; h0 input

function u = fhan(e, v2, r0, h0)

d = r0*h0^2;
a0 = h0*v2;
y = e + a0;

a1 = sqrt(d*(d + 8*abs(y)));
a2 = a0 + sign(y)*(a1 - d)/2;

sy = (sign(y + d) - sign(y - d))/2;
a = (a0 + y - a2)*sy + a2;

sa = (sign(a + d) - sign(a - d))/2;

u = -r0*(a/d - sign(a))*sa - r0*sign(a);

end

== matlab function adrc_pid/Quad Dynamics2/Subsystem/MATLAB Function2 ==
  data: phi input size=1; phidot output size=1; theta input size=1; p input size=1; q input size=1; r input size=1; U input; inertia_mx input; pdot output size=1
function [phidot, pdot] = roll_dynamics( ...
    phi, theta, p, q, r, U, inertia_mx)

Ix = inertia_mx(1);
Iy = inertia_mx(2);
Iz = inertia_mx(3);

tau_roll = U(2);

phidot = p + sin(phi)*tan(theta)*q ...
           + cos(phi)*tan(theta)*r;

pdot = (tau_roll + (Iy-Iz)*q*r)/Ix;

end

== matlab function adrc_pid/Quad Dynamics2/Subsystem/MATLAB Function3 ==
  data: phi input size=1; thetadot output size=1; p input size=1; q input size=1; r input size=1; U input size=[4 1]; inertia_mx input size=[3 1]; qdot output size=1
function [thetadot, qdot] = pitch_dynamics( ...
    phi, p, q, r, U, inertia_mx)

Ix = inertia_mx(1);
Iy = inertia_mx(2);
Iz = inertia_mx(3);

tau_pitch = U(3);

thetadot = cos(phi)*q - sin(phi)*r;

qdot = (tau_pitch + (Iz-Ix)*p*r)/Iy;

end

== matlab function adrc_pid/Quad Dynamics2/Subsystem/MATLAB Function4 ==
  data: phi input size=1; psidot output size=1; theta input size=1; p input size=1; q input size=1; r input size=1; U input; inertia_mx input; rdot output size=1
function [psidot, rdot] = yaw_dynamics( ...
    phi, theta, p, q, r, U, inertia_mx)

Ix = inertia_mx(1);
Iy = inertia_mx(2);
Iz = inertia_mx(3);

psidot = 0;
rdot = 0;

tau_yaw = U(4);

psidot = (sin(phi)*q + cos(phi)*r)/cos(theta);

rdot = (tau_yaw + (Ix-Iy)*p*q)/Iz;

end

== matlab function adrc_pid/Quad Dynamics1/Subsystem/MATLAB Function ==
  data: U input; phi input; xdd output; theta input; psi input; Fx input; m input
function xdd = x_dynamics(U, phi, theta, psi, Fx, m)

T = U(1);
xdd = (T/m)*(cos(psi)*sin(theta)*cos(phi) ...
               + sin(psi)*sin(phi)) + Fx/m;

end

== matlab function adrc_pid/Quad Dynamics2/Subsystem/z_dynamics/c_calc ==
  data: z input; c output; h input
function c = fcn(z, h)

if z > h/2
    c = 0;
elseif z < -h/2
    c = h;
else 
    c = h/2 - z;
end

== matlab function adrc_pid/Quad Dynamics1/Subsystem/MATLAB Function1 ==
  data: U input; ydd output; phi input; theta input; psi input; Fy input; m input
function ydd = y_dynamics(U, phi, theta, psi, Fy, m)

T = U(1);

ydd = (T/m)*(sin(psi)*sin(theta)*cos(phi) ...
               - cos(psi)*sin(phi)) + Fy/m;

end

== matlab function adrc_pid/Quad Dynamics1/Subsystem/MATLAB Function2 ==
  data: phi input size=1; phidot output size=1; theta input size=1; p input size=1; q input size=1; r input size=1; U input; inertia_mx input; pdot output size=1
function [phidot, pdot] = roll_dynamics( ...
    phi, theta, p, q, r, U, inertia_mx)

Ix = inertia_mx(1);
Iy = inertia_mx(2);
Iz = inertia_mx(3);

tau_roll = U(2);

phidot = p + sin(phi)*tan(theta)*q ...
           + cos(phi)*tan(theta)*r;

pdot = (tau_roll + (Iy-Iz)*q*r)/Ix;

end

== matlab function adrc_pid/Quad Dynamics1/Subsystem/MATLAB Function3 ==
  data: phi input size=1; thetadot output size=1; p input size=1; q input size=1; r input size=1; U input size=[4 1]; inertia_mx input size=[3 1]; qdot output size=1
function [thetadot, qdot] = pitch_dynamics( ...
    phi, p, q, r, U, inertia_mx)

Ix = inertia_mx(1);
Iy = inertia_mx(2);
Iz = inertia_mx(3);

tau_pitch = U(3);

thetadot = cos(phi)*q - sin(phi)*r;

qdot = (tau_pitch + (Iz-Ix)*p*r)/Iy;

end

== matlab function adrc_pid/Quad Dynamics1/Subsystem/MATLAB Function4 ==
  data: phi input size=1; psidot output size=1; theta input size=1; p input size=1; q input size=1; r input size=1; U input; inertia_mx input; rdot output size=1
function [psidot, rdot] = yaw_dynamics( ...
    phi, theta, p, q, r, U, inertia_mx)

Ix = inertia_mx(1);
Iy = inertia_mx(2);
Iz = inertia_mx(3);

psidot = 0;
rdot = 0;

tau_yaw = U(4);

psidot = (sin(phi)*q + cos(phi)*r)/cos(theta);

rdot = (tau_yaw + (Ix-Iy)*p*q)/Iz;

end

== matlab function adrc_pid/Quad Dynamics1/Subsystem/z_dynamics/c_calc ==
  data: z input; c output; h input
function c = fcn(z, h)

if z > h/2
    c = 0;
elseif z < -h/2
    c = h;
else 
    c = h/2 - z;
end

== matlab function adrc_pid/Quad Dynamics2/Subsystem/MATLAB Function ==
  data: U input; phi input; xdd output; theta input; psi input; Fx input; m input
function xdd = x_dynamics(U, phi, theta, psi, Fx, m)

T = U(1);
xdd = (T/m)*(cos(psi)*sin(theta)*cos(phi) ...
               + sin(psi)*sin(phi)) + Fx/m;

end
